simulink model "TestingFile1"  (R2022b)
settings: Solver=VariableStepAuto  StartTime=0.0  StopTime=24  FixedStep=5e-9  MaxStep=0.01  RelTol=1e-3  AbsTol=1e-6
undefined symbols (not defined in the file): Acid, Lead
libraries: spsSeriesRLCBranchLib x24, spsCurrentMeasurementLib x19, spsIdealSwitchLib x10, spsMosfetLib x6, spsPWMGeneratorDCDCLib x5, spsDiodeLib x4, spsBatteryLib x2, slpidlib x2, spsIGBTLib x2, spsPVArrayLib x2, spsVoltageMeasurementLib x2, spspowerguiLib x1
(part 1 of 2)
settings Model: Creator=Haroon  LastModifiedBy=Haroon

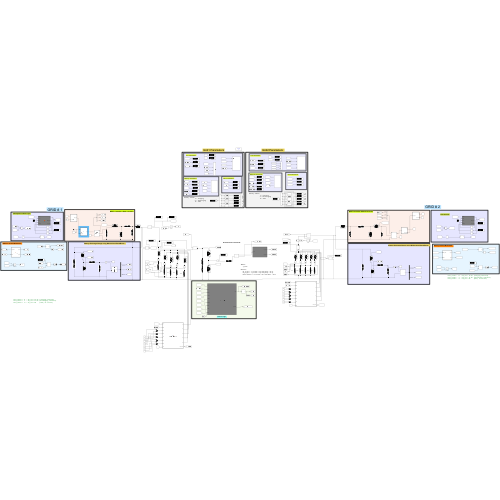
[thumbnail: Simulink's stored preview of the top-level diagram]
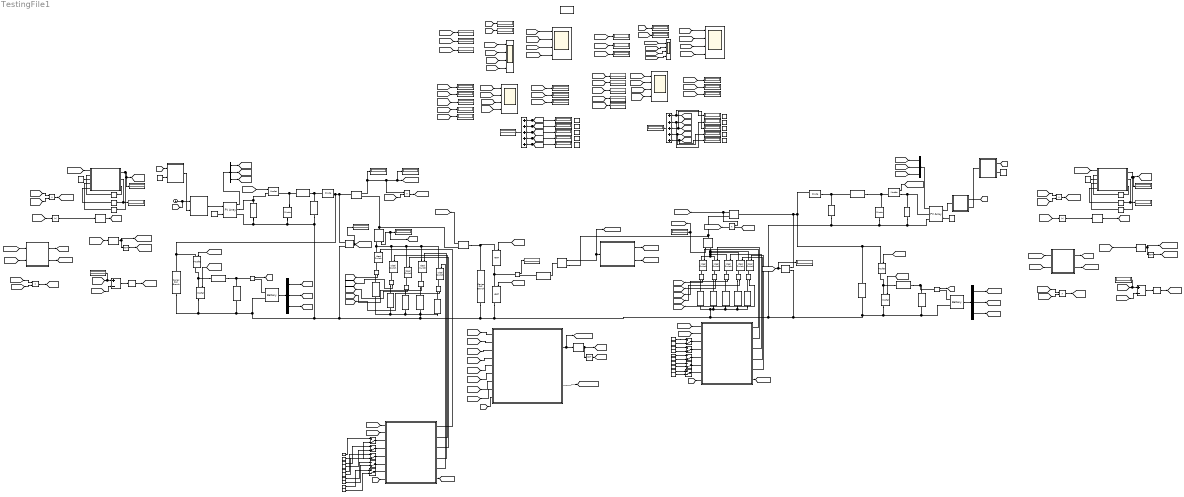
== system TestingFile1 ==
  note: Battery Status:
      | 1 = Charging
      | -1 = Discharging
      | 0 = Idle
  note: INPUTS:
      | I_flow
      |
      | OUTPUTS:
      | G1_to_G2 = 1 [I-flow > 0] and [Duty > 0.5]
      | G2_to_G1 = 1 [I-flow < 0] and [Duty < 0.5]
      | Both outputs = 0 [I-flow = 0] and [Duty = 0.5]
  note: batt_status = +1 → Vb_ref = 14.4V (charging reference)
      | batt_status = -1 → Vb_ref = 11.0V (discharging reference)
      | batt_status = 0 → Ib_ref = 0A (idle, no current)
  note: GRID # 1
  note: Control Logic
  note: Biredictional converter
  note: MPPT Controller - Buck converter
  note: Battery's Control Mechanism
  note: Battery Discharge/Charge using Bidirectional Buck/Boost Converter
  note: PV1 Parameters
  note: P&O Algorithm / MPPT Logic
  note: Battery1 Parameters
  note: Bus1 Parameters
  note: P&O Algorithm
  note: Battery2 Parameters
  note: PV2 Parameters
  note: Bus2 Parameters
  note: GRID # 2
  note: Grid1 Parameters
  note: Grid2 Parameters
  note: Battery's Control Mechanism
  note: batt_status = +1 → Vb_ref = 14.4V (charging reference)
      | batt_status = -1 → Vb_ref = 11.0V (discharging reference)
      | batt_status = 0 → Ib_ref = 0A (idle, no current)
  note: Battery Status:
      | 1 = Charging
      | -1 = Discharging
      | 0 = Idle
  note: Battery Discharge/Charge using Bidirectional Buck/Boost Converter
  note: MPPT Controller & Buck converter
  Abs : Abs  SaturateOnIntegerOverflow=off
  Abs2 : Abs  SaturateOnIntegerOverflow=off
  Add1 : Sum  Inputs=+-
  Add2 : Sum  Inputs=+++++
  Add3 : Sum  Inputs=+++++
  Add4 : Sum  Inputs=+-
  Battery : spsBatteryLib/Battery  BatType=Lead-Acid  ShowTempParam=off  ThermalPreset=no  ShowAgeParam=off  NomV=12  NomQ=0.01389  SOC=70  Batt_Tr=0.5  PresetModel=off  MaxQ=0.01389  MinV=10.5  FullV=14.4  Dis_rate=5  R=0.1  Normal_OP=0.01389  expZone="[12.2     0.001389]"  current=[6.5 13 32.5]  Units=Time  Tci=20  NomT=20  T2=-30  MaxQ2=4.8  FullV2=7.1  Normal_OP2=5.655  expZone2="[6.58           1]"  Rca=0.6  ti=2000  Dp=0  Neq0=0  Tsim=1e6  Ta1=25  Qeol=5.4*0.9  Reol=0.013333*1.2  Char_age=[2.3478, 3]  Dis_age=[2.3478, 10]  N1=1500  N2=10500  N3=1000  N4=1400  Ta2=45  N5=950
  Battery1 : spsBatteryLib/Battery  BatType=Lead-Acid  ShowTempParam=off  ThermalPreset=no  ShowAgeParam=off  NomV=12  NomQ=0.01389  SOC=70  Batt_Tr=0.5  PresetModel=off  MaxQ=0.01389  MinV=10.5  FullV=14.4  Dis_rate=5  R=0.1  Normal_OP=0.01389  expZone="[12.2     0.001389]"  current=[6.5 13 32.5]  Units=Time  Tci=20  NomT=20  T2=-30  MaxQ2=4.8  FullV2=7.1  Normal_OP2=5.655  expZone2="[6.58           1]"  Rca=0.6  ti=2000  Dp=0  Neq0=0  Tsim=1e6  Ta1=25  Qeol=5.4*0.9  Reol=0.013333*1.2  Char_age=[2.3478, 3]  Dis_age=[2.3478, 10]  N1=1500  N2=10500  N3=1000  N4=1400  Ta2=45  N5=950
  Bus Selector : BusSelector  OutputSignals=Current (A),Voltage (V),SOC (%)
  Bus Selector1 : BusSelector  OutputSignals=V_PV,I_PV,Irradiance (W/m2)
  Bus Selector2 : BusSelector  OutputSignals=V_PV,I_PV,Irradiance (W/m2)
  Bus Selector3 : BusSelector  OutputSignals=Current (A),Voltage (V),SOC (%)
  Clock : Clock
  Constant{1,5,10,12,14,16..17,19,21,24} (10 alike) : Constant  Value=0
  Constant{4,6,11,13,15,18,20,22..23,25} (10 alike) : Constant
  Constant2 : Constant  Value=25
  Constant7 : Constant  Value=25
  Constant8 : Constant  Value=1000
  Constant9 : Constant  Value=1000
  Current Measurement{,1..18} (19 alike) : spsCurrentMeasurementLib/Current Measurement  PhasorSimulation=off  OutputType=Complex  PSBequivalent=0
  Diode{,1..3} (4 alike) : spsDiodeLib/Diode  Ron=0.001  Lon=0  Vf=0.8  IC=0  UseSnubber=0  Rs=500  Cs=250e-9  Measurements=on
  Discrete PID Controller1 : slpidlib/PID Controller  Controller=PI  Form=Parallel  TimeDomain=Discrete-time  UseExternalTs=off  SampleTime=50e-6  IntegratorMethod=Forward Euler  FilterMethod=Forward Euler  ControllerParametersSource=internal  P=0.3  I=0.03  UseKiTs=off  D=0  N=100  UseFilter=on  TunerSelectOption=Transfer Function Based (PID Tuner App)  InitialConditionSource=internal  InitialConditionForIntegrator=0.5  InitialConditionForFilter=0  DifferentiatorICPrevScaledInput=0  ExternalReset=none  TrackingMode=off  Kt=1  LimitOutput=on  SatLimitsSource=internal  UpperSaturationLimit=0.95  LowerSaturationLimit=0.05  LinearizeAsGain=on  AntiWindupMode=back-calculation  Kb=1  LimitIntegrator=off  UpperIntegratorSaturationLimit=inf  LowerIntegratorSaturationLimit=-inf  POutMin=[]  POutMax=[]  IOutMin=[]  IOutMax=[]  DOutMin=[]  DOutMax=[]  NOutMin=[]  NOutMax=[]  SumOutMin=[]  SumOutMax=[]  SaturationOutMin=[]  SaturationOutMax=[]  PParamMin=[]  PParamMax=[]  IParamMin=[]  IParamMax=[]  DParamMin=[]  DParamMax=[]  NParamMin=[]  NParamMax=[]  KbParamMin=[]  KbParamMax=[]  KtParamMin=[]  KtParamMax=[]  KbOutMin=[]  KbOutMax=[]  KtOutMin=[]  KtOutMax=[]  IntegratorOutMin=[]  IntegratorOutMax=[]  FilterOutMin=[]  FilterOutMax=[]  SumI1OutMin=[]  SumI1OutMax=[]  SumI2OutMin=[]  SumI2OutMax=[]  SumI3OutMin=[]  SumI3OutMax=[]  SumI4OutMin=[]  SumI4OutMax=[]  SumDOutMin=[]  SumDOutMax=[]  DifferentiatorOutMin=[]  DifferentiatorOutMax=[]  FilterDiffOutCoefMin=[]  FilterDiffOutCoefMax=[]  ReciprocalOutMin=[]  ReciprocalOutMax=[]  SumDenOutMin=[]  SumDenOutMax=[]  SumNumOutMin=[]  SumNumOutMax=[]  DivideOutMin=[]  DivideOutMax=[]  UdiffTsProdOutMin=[]  UdiffTsProdOutMax=[]  NTsProdOutMin=[]  NTsProdOutMax=[]  UintegralTsProdOutMin=[]  UintegralTsProdOutMax=[]  UngainTsProdOutMin=[]  UngainTsProdOutMax=[]  ClampingZeroOutDataTypeStr=Inherit: Inherit via back propagation  ClampingZeroOutMin=[]  ClampingZeroOutMax=[]  FilterDenConstantOutDataTypeStr=Inherit: Inherit via back propagation  FilterDenConstantOutMin=[]  FilterDenConstantOutMax=[]  PCopyOutDataTypeStr=Inherit: Inherit via back propagation  PCopyOutMin=[]  PCopyOutMax=[]  NCopyOutDataTypeStr=Inherit: Inherit via back propagation  NCopyOutMin=[]  NCopyOutMax=[]  IntegratorContinuousStateAttributes=''  IntegratorStateMustResolveToSignalObject=off  IntegratorRTWStateStorageClass=Auto  FilterContinuousStateAttributes=''  FilterStateMustResolveToSignalObject=off  FilterRTWStateStorageClass=Auto  ParallelPVariant=InternalParameters  IdealPVariant=Disabled  IVariant=InternalParameters  DVariant=Disabled  IntegratorVariant=Discrete  SatVariant=Enabled  AWVariant=BackCalculation  PCopyVariant=Disabled  TRVariant=Disabled  FdbkBlocksVariant=Forward  IdealPFdbkVariant=Disabled  SatFdbkVariant=Disabled  DerivativeFilterVariant=Disabled  NVariant=Disabled  NCopyVariant=Disabled_SignalSpec  FilterICVariant=Disabled  IntegratorICVariant=InternalICs  ExternalResetVariant=Disabled  TRSumVariant=Passthrough  SumFdbkVariant=Disabled  SumVariant=Sum_PI  TsampFilterVariant=InternalTs  TsampNgainVariant=Passthrough  TsampIntegralVariant=Passthrough  ExternalSaturationOutDataTypeStr=Inherit: Same as second input
      settings: LibrarySourceBlock=simulink/Discrete/Discrete PID Controller
  Discrete PID Controller4 : slpidlib/PID Controller  Controller=PI  Form=Parallel  TimeDomain=Discrete-time  UseExternalTs=off  SampleTime=50e-6  IntegratorMethod=Forward Euler  FilterMethod=Forward Euler  ControllerParametersSource=internal  P=0.3  I=0.03  UseKiTs=off  D=0  N=100  UseFilter=on  TunerSelectOption=Transfer Function Based (PID Tuner App)  InitialConditionSource=internal  InitialConditionForIntegrator=0.5  InitialConditionForFilter=0  DifferentiatorICPrevScaledInput=0  ExternalReset=none  TrackingMode=off  Kt=1  LimitOutput=on  SatLimitsSource=internal  UpperSaturationLimit=0.95  LowerSaturationLimit=0.05  LinearizeAsGain=off  AntiWindupMode=back-calculation  Kb=1  LimitIntegrator=on  UpperIntegratorSaturationLimit=Inf  LowerIntegratorSaturationLimit=-Inf  POutMin=[]  POutMax=[]  IOutMin=[]  IOutMax=[]  DOutMin=[]  DOutMax=[]  NOutMin=[]  NOutMax=[]  SumOutMin=[]  SumOutMax=[]  SaturationOutMin=[]  SaturationOutMax=[]  PParamMin=[]  PParamMax=[]  IParamMin=[]  IParamMax=[]  DParamMin=[]  DParamMax=[]  NParamMin=[]  NParamMax=[]  KbParamMin=[]  KbParamMax=[]  KtParamMin=[]  KtParamMax=[]  KbOutMin=[]  KbOutMax=[]  KtOutMin=[]  KtOutMax=[]  IntegratorOutMin=[]  IntegratorOutMax=[]  FilterOutMin=[]  FilterOutMax=[]  SumI1OutMin=[]  SumI1OutMax=[]  SumI2OutMin=[]  SumI2OutMax=[]  SumI3OutMin=[]  SumI3OutMax=[]  SumI4OutMin=[]  SumI4OutMax=[]  SumDOutMin=[]  SumDOutMax=[]  DifferentiatorOutMin=[]  DifferentiatorOutMax=[]  FilterDiffOutCoefMin=[]  FilterDiffOutCoefMax=[]  ReciprocalOutMin=[]  ReciprocalOutMax=[]  SumDenOutMin=[]  SumDenOutMax=[]  SumNumOutMin=[]  SumNumOutMax=[]  DivideOutMin=[]  DivideOutMax=[]  UdiffTsProdOutMin=[]  UdiffTsProdOutMax=[]  NTsProdOutMin=[]  NTsProdOutMax=[]  UintegralTsProdOutMin=[]  UintegralTsProdOutMax=[]  UngainTsProdOutMin=[]  UngainTsProdOutMax=[]  ClampingZeroOutDataTypeStr=Inherit: Inherit via back propagation  ClampingZeroOutMin=[]  ClampingZeroOutMax=[]  FilterDenConstantOutDataTypeStr=Inherit: Inherit via back propagation  FilterDenConstantOutMin=[]  FilterDenConstantOutMax=[]  PCopyOutDataTypeStr=Inherit: Inherit via back propagation  PCopyOutMin=[]  PCopyOutMax=[]  NCopyOutDataTypeStr=Inherit: Inherit via back propagation  NCopyOutMin=[]  NCopyOutMax=[]  IntegratorContinuousStateAttributes=''  IntegratorStateMustResolveToSignalObject=off  IntegratorRTWStateStorageClass=Auto  FilterContinuousStateAttributes=''  FilterStateMustResolveToSignalObject=off  FilterRTWStateStorageClass=Auto  ParallelPVariant=InternalParameters  IdealPVariant=Disabled  IVariant=InternalParameters  DVariant=Disabled  IntegratorVariant=Discrete  SatVariant=Enabled  AWVariant=BackCalculation  PCopyVariant=Disabled  TRVariant=Disabled  FdbkBlocksVariant=Forward  IdealPFdbkVariant=Disabled  SatFdbkVariant=Disabled  DerivativeFilterVariant=Disabled  NVariant=Disabled  NCopyVariant=Disabled_SignalSpec  FilterICVariant=Disabled  IntegratorICVariant=InternalICs  ExternalResetVariant=Disabled  TRSumVariant=Passthrough  SumFdbkVariant=Disabled  SumVariant=Sum_PI  TsampFilterVariant=InternalTs  TsampNgainVariant=Passthrough  TsampIntegralVariant=Passthrough  ExternalSaturationOutDataTypeStr=Inherit: Same as second input
      settings: LibrarySourceBlock=simulink/Discrete/Discrete PID Controller
  Display{,1..5,8..16,18..19,21..31,36..48} (41 alike) : Display
  Goto29 : Goto
  IGBT2 : spsIGBTLib/IGBT  Ron=0.001  Lon=0  Vf=1  Tf=1e-6  Tt=2e-6  IC=0  Rs=1e5  Cs=inf  Measurements=on
  IGBT3 : spsIGBTLib/IGBT  Ron=0.001  Lon=0  Vf=1  Tf=1e-6  Tt=2e-6  IC=0  Rs=1e5  Cs=inf  Measurements=on
  I_PV : Display
  I_PV1 : Display
  Ideal Switch{,1..9} (10 alike) : spsIdealSwitchLib/Ideal Switch  Ron=0.001  Lon=0  IC=0  Rs=1e5  Cs=inf  Measurements=on
  Irradiance : Display
  Irradiance1 : Display
  Lamp{1..10} (10 alike) : LampBlock  LabelPosition=Hide
  Logical Operator : Logic  Operator=NOT  AllPortsSameDT=off  OutDataTypeStr=boolean
  Logical Operator2 : Logic  Operator=NOT  AllPortsSameDT=off  OutDataTypeStr=boolean
  Logical Operator3 : Logic  Operator=NOT  AllPortsSameDT=off  OutDataTypeStr=boolean
  MATLAB Function : MATLAB Function  TreatAsAtomicUnit=on
  MATLAB Function1 : MATLAB Function  TreatAsAtomicUnit=on
  MATLAB Function10 : MATLAB Function  TreatAsAtomicUnit=on
  MATLAB Function11 : MATLAB Function  TreatAsAtomicUnit=on
  MATLAB Function2 : MATLAB Function  TreatAsAtomicUnit=on
  MATLAB Function3 : MATLAB Function  TreatAsAtomicUnit=on
  MATLAB Function4 : MATLAB Function  TreatAsAtomicUnit=on
  MATLAB Function5 : MATLAB Function  TreatAsAtomicUnit=on
  MATLAB Function6 : MATLAB Function  TreatAsAtomicUnit=on
  MATLAB Function7 : MATLAB Function  TreatAsAtomicUnit=on
  MATLAB Function8 : MATLAB Function  TreatAsAtomicUnit=on
  MATLAB Function9 : MATLAB Function  TreatAsAtomicUnit=on
  Manual Switch{,1..9} (10 alike) : ManualSwitch  CurrentSetting=0
  Memory{,1,3..4} (4 alike) : Memory
  Memory2 : Memory  InitialCondition=0.5
  Memory5 : Memory  InitialCondition=0.5
  Mosfet{,1..5} (6 alike) : spsMosfetLib/Mosfet  Ron=0.1  Lon=0  Rd=0.01  Vfd=0  IC=0  Rs=1e5  Cs=inf  Measurements=on
  PV Array : spsPVArrayLib/PV Array  Npar=1  Nser=1  PlotType=array @ 25 deg.C & specified irradiances  S_vec="[ 1000  500  100 0 ]"  Temp_C_vec="[ 45 25  ]"  ModuleName=User-defined  PlotWhenSelected=off  Pm=262.6404  Ncell=72  Voc=26.7  Isc=13.97  Vm=22.22  Im=11.82  beta_Voc_pc=-0.37  alpha_Isc_pc=0.06  beta_Voc=-0.09879  alpha_Isc=0.008382  IL=14.0891  I0=6.4727e-10  nI=0.61024  Rsh=13.454  Rs=0.082721  RobustModel=off  RobustCellTemperature=313.3991  BAL=on  Tc=1e-6  Tfilter=5e-5
  PV Array1 : spsPVArrayLib/PV Array  Npar=1  Nser=1  PlotType=array @ 1000 W/m2 & specified temperatures  S_vec="[ 1000  500  100 ]"  Temp_C_vec="[ 45 25  ]"  ModuleName=User-defined  PlotWhenSelected=off  Pm=262.6404  Ncell=72  Voc=26.7  Isc=13.97  Vm=22.22  Im=11.82  beta_Voc_pc=-0.355  alpha_Isc_pc=0.06  beta_Voc=-0.094785  alpha_Isc=0.008382  IL=14.0358  I0=3.7786e-10  nI=0.59666  Rsh=13.8554  Rs=0.087929  RobustModel=off  RobustCellTemperature=313.3991  BAL=on  Tc=1e-6  Tfilter=5e-5
  PWM Generator (DC-DC) : spsPWMGeneratorDCDCLib/PWM Generator (DC-DC)  Fsw=5000  Ts=0
  PWM Generator (DC-DC)1 : spsPWMGeneratorDCDCLib/PWM Generator (DC-DC)  Fsw=20000  Ts=0
  PWM Generator (DC-DC)2 : spsPWMGeneratorDCDCLib/PWM Generator (DC-DC)  Fsw=5000  Ts=0
  PWM Generator (DC-DC)3 : spsPWMGeneratorDCDCLib/PWM Generator (DC-DC)  Fsw=20000  Ts=0
  PWM Generator (DC-DC)5 : spsPWMGeneratorDCDCLib/PWM Generator (DC-DC)  Fsw=5000  Ts=0
  P_Bus2 : Product
  P_PV : Display
  P_PV1 : Display
  P_battery1 : Product
  P_battery2 : Product
  P_bus1 : Product
  Ppv1 : Product
  Ppv2 : Product
  Pulse Generator : DiscretePulseGenerator  PulseType=Time based  Period=0.005  PulseWidth=99.9999
  Pulse Generator1 : DiscretePulseGenerator  PulseType=Time based  Period=0.005  PulseWidth=99.9999
  Scope{,1..5} (6 alike) : Scope  NumInputPorts=4
  Series RLC Branch : spsSeriesRLCBranchLib/Series RLC Branch  LConnTagsString=__new0  RConnTagsString=__new0  BranchType=RC  Resistance=1e-4  Inductance=1e-3  SetiL0=off  InitialCurrent=0  Capacitance=680e-6  Setx0=off  InitialVoltage=0  Measurements=None
  Series RLC Branch1 : spsSeriesRLCBranchLib/Series RLC Branch  LConnTagsString=__new0  RConnTagsString=__new0  BranchType=RL  Resistance=1e-4  Inductance=13e-3  SetiL0=off  InitialCurrent=0  Capacitance=1e-6  Setx0=off  InitialVoltage=0  Measurements=None
  Series RLC Branch11 : spsSeriesRLCBranchLib/Series RLC Branch  LConnTagsString=__new0  RConnTagsString=__new0  BranchType=RC  Resistance=1e-4  Inductance=1e-3  SetiL0=off  InitialCurrent=0  Capacitance=1000e-6  Setx0=off  InitialVoltage=0  Measurements=None
  Series RLC Branch12 : spsSeriesRLCBranchLib/Series RLC Branch  LConnTagsString=__new0  RConnTagsString=__new0  BranchType=RL  Resistance=1e-4  Inductance=13e-3  SetiL0=off  InitialCurrent=0  Capacitance=1e-6  Setx0=off  InitialVoltage=0  Measurements=None
  Series RLC Branch13 : spsSeriesRLCBranchLib/Series RLC Branch  LConnTagsString=__new0  RConnTagsString=__new0  BranchType=RC  Resistance=1e-4  Inductance=1e-3  SetiL0=off  InitialCurrent=0  Capacitance=20e-6  Setx0=off  InitialVoltage=0  Measurements=None
  Series RLC Branch14 : spsSeriesRLCBranchLib/Series RLC Branch  LConnTagsString=__new0  RConnTagsString=__new0  BranchType=RL  Resistance=1  Inductance=1e-3  SetiL0=off  InitialCurrent=0  Capacitance=1e-6  Setx0=off  InitialVoltage=0  Measurements=None
  Series RLC Branch2 : spsSeriesRLCBranchLib/Series RLC Branch  LConnTagsString=__new0  RConnTagsString=__new0  BranchType=RC  Resistance=1e-4  Inductance=1e-3  SetiL0=off  InitialCurrent=0  Capacitance=100e-6  Setx0=off  InitialVoltage=0  Measurements=None
  Series RLC Branch24 : spsSeriesRLCBranchLib/Series RLC Branch  LConnTagsString=__new0  RConnTagsString=__new0  BranchType=RL  Resistance=0.01  Inductance=24e-6  SetiL0=off  InitialCurrent=0  Capacitance=1e-6  Setx0=off  InitialVoltage=0  Measurements=None
  Series RLC Branch3 : spsSeriesRLCBranchLib/Series RLC Branch  LConnTagsString=__new0  RConnTagsString=__new0  BranchType=RC  Resistance=0.001  Inductance=1e-3  SetiL0=off  InitialCurrent=0  Capacitance=400e-6  Setx0=off  InitialVoltage=0  Measurements=None
  Series RLC Branch4 : spsSeriesRLCBranchLib/Series RLC Branch  LConnTagsString=__new0  RConnTagsString=__new0  BranchType=RL  Resistance=0.01  Inductance=24e-6  SetiL0=off  InitialCurrent=0  Capacitance=1e-6  Setx0=off  InitialVoltage=0  Measurements=None
  Series RLC Branch5 : spsSeriesRLCBranchLib/Series RLC Branch  LConnTagsString=__new0  RConnTagsString=__new0  BranchType=RC  Resistance=0.01  Inductance=1e-3  SetiL0=off  InitialCurrent=0  Capacitance=97e-6  Setx0=off  InitialVoltage=0  Measurements=None
  Series RLC Branch6 : spsSeriesRLCBranchLib/Series RLC Branch  LConnTagsString=__new0  RConnTagsString=__new0  BranchType=RC  Resistance=1  Inductance=1e-3  SetiL0=off  InitialCurrent=0  Capacitance=1e-6  Setx0=off  InitialVoltage=0  Measurements=None
  Series RLC Branch7 : spsSeriesRLCBranchLib/Series RLC Branch  LConnTagsString=__new0  RConnTagsString=__new0  BranchType=RC  Resistance=0.001  Inductance=1e-3  SetiL0=off  InitialCurrent=0  Capacitance=400e-6  Setx0=off  InitialVoltage=0  Measurements=None
  Series RLC Branch9 : spsSeriesRLCBranchLib/Series RLC Branch  LConnTagsString=__new0  RConnTagsString=__new0  BranchType=RC  Resistance=0.01  Inductance=1e-3  SetiL0=off  InitialCurrent=0  Capacitance=97e-6  Setx0=off  InitialVoltage=0  Measurements=None
  Stage : Display
  Stage1 : Display
  V_PV : Display
  V_PV1 : Display
  Voltage Measurement : spsVoltageMeasurementLib/Voltage Measurement  PhasorSimulation=off  OutputType=Complex  PSBequivalent=0
  Voltage Measurement1 : spsVoltageMeasurementLib/Voltage Measurement  PhasorSimulation=off  OutputType=Complex  PSBequivalent=0
  bulb{11..12,21..22} (4 alike) : spsSeriesRLCBranchLib/Series RLC Branch  LConnTagsString=__new0  RConnTagsString=__new0  BranchType=R  Resistance=7.2  Inductance=1e-3  SetiL0=off  InitialCurrent=0  Capacitance=1e-6  Setx0=off  InitialVoltage=0  Measurements=None
  fan{11..12,21..22} (4 alike) : spsSeriesRLCBranchLib/Series RLC Branch  LConnTagsString=__new0  RConnTagsString=__new0  BranchType=R  Resistance=2.4  Inductance=1e-3  SetiL0=off  InitialCurrent=0  Capacitance=1e-6  Setx0=off  InitialVoltage=0  Measurements=None
  powergui : spspowerguiLib/powergui  Priority=1  SimulationMode=Discrete  SampleTime=1  frequency=60  Iterations=50  frequencyindice=0  Pbase=100e6  ErrMax=1e-4  UnitsV=kV  UnitsW=MW  buscounter=0  FunctionMessages=off  echomessages=off  EnableUseOfTLC=off  CurrentSourceSwitches=off  DisableSnubberDevices=off  DisableRonSwitches=off  DisableVfSwitches=off  DisplayEquations=off  AutomaticDiscreteSolvers=off  SolverType=Tustin/Backward Euler (TBE)  Interpol=off  ExternalGateDelay=off  methode=off  Ts=100  x0status=blocks  SPID=on  SwTol=0  HookPort=off  NonlinearTolerance=1e-4  nMaxIteration=100  ContinueOnMaxIteration=off  RestoreLinks=warning  ResistiveCurrentMeasurement=off  Frange=[0:2:500]  Ylog=off  Xlog=on  ShowGrid=off  save=off  variable=ZData  structure=0  ZoomFFT=off  StartTime=0.0  cycles=1  DisplayStyle=1  fundamental=60  FreqAxis=off  MaxFrequency=1000  frequencyindicesteady=1  RmsSteady=1  display=off
  pump : spsSeriesRLCBranchLib/Series RLC Branch  LConnTagsString=__new0  RConnTagsString=__new0  BranchType=R  Resistance=1.44  Inductance=1e-3  SetiL0=off  InitialCurrent=0  Capacitance=1e-6  Setx0=off  InitialVoltage=0  Measurements=None
  pump1 : spsSeriesRLCBranchLib/Series RLC Branch  LConnTagsString=__new0  RConnTagsString=__new0  BranchType=R  Resistance=1.44  Inductance=1e-3  SetiL0=off  InitialCurrent=0  Capacitance=1e-6  Setx0=off  InitialVoltage=0  Measurements=None
  wires:
  [Vpv_Grid1] -> Ppv1/1
  MATLAB Function/3(Pold_out) -> Memory/1
  MATLAB Function/2(Stage_out) -> Stage/1, Memory1/1
  Memory/1 -> MATLAB Function/2(P_old)
  [Ipv_Grid1] -> Ppv1/2
  Current Measurement/1 -> [I_bat1]
  PV Array/1 -> Bus Selector1/1
  MATLAB Function/1(Y) -> Memory2/1, [d_Grid1], Display4/1
  Ppv1/1 -> [P_new_Grid1]
  Pulse Generator/1 -> MATLAB Function/3(Delay)
  [SOC_Grid1] -> Display2/1
  [Vpv_Grid1] -> V_PV/1
  Memory2/1 -> MATLAB Function/4(Yin)
  [P_new_Grid1] -> P_PV/1
  [Ipv_Grid1] -> I_PV/1
  Battery/1 -> Bus Selector/1
  Constant2/1 -> PV Array/2
  Bus Selector1/1 -> [Vpv_Grid1]  "<V_PV>"
  [vb_Grid1] -> Display/1
  Bus Selector1/2 -> [Ipv_Grid1]  "<I_PV>"
  Bus Selector/3 -> [SOC_Grid1]  "<SOC (%)>"
  Bus Selector/2 -> [vb_Grid1]  "<Voltage (V)>"
  Bus Selector/1 -> [ib_Grid1]  "<Current (A)>"
  Memory1/1 -> MATLAB Function/5(Stage_in)
  [ib_Grid1] -> Display1/1
  Bus Selector2/1 -> [Vpv_Grid2]  "<V_PV>"
  Constant7/1 -> PV Array1/2
  PV Array1/1 -> Bus Selector2/1
  Bus Selector2/2 -> [Ipv_Grid2]  "<I_PV>"
  Bus Selector3/1 -> [ib_Grid2]  "<Current (A)>"
  Bus Selector3/3 -> [SOC_Grid2]  "<SOC (%)>"
  Current Measurement1/1 -> [I_bat2]
  Bus Selector3/2 -> [vb_Grid2]  "<Voltage (V)>"
  Battery1/1 -> Bus Selector3/1
  Current Measurement2/1 -> Display10/1, [I_boost_Grid1], P_bus1/1, Display11/1
  P_bus1/1 -> [PLoad_Grid1]
  Current Measurement3/1 -> [I1_total], Display3/1
  Current Measurement4/1 -> Goto29/1
  Current Measurement5/1 -> Display5/1
  [s_p_Grid_X] -> IGBT2/1
  [s_n_Grid_X] -> IGBT3/1
  Current Measurement6/1 -> [I_Grid1_to_Grid2], MATLAB Function1/1(I_flow)
  MATLAB Function1/2(G2_to_G1) -> [Grid2to1]
  MATLAB Function1/1(G1_to_G2) -> [Grid1to2]
  Current Measurement7/1 -> [I2_total], Display8/1
  Current Measurement8/1 -> [I_boost_Grid2], P_Bus2/1
  P_Bus2/1 -> [PLoad_Grid2]
  [P_new_Grid1] -> MATLAB Function/1(P_new)
  [I_boost_Grid1] -> Display14/1
  [V_bus_Grid1] -> Display13/1
  [PLoad_Grid1] -> Display15/1
  Memory4/1 -> MATLAB Function3/5(Stage_in)
  Memory5/1 -> MATLAB Function3/4(Yin)
  [d_Grid2] -> Abs2/1
  Ppv2/1 -> [P_new_Grid2]
  MATLAB Function3/1(Y) -> Memory5/1, [d_Grid2], Display16/1
  Memory3/1 -> MATLAB Function3/2(P_old)
  Pulse Generator1/1 -> MATLAB Function3/3(Delay)
  [Ipv_Grid2] -> Ppv2/2
  [Vpv_Grid2] -> Ppv2/1
  MATLAB Function3/3(Pold_out) -> Memory3/1
  MATLAB Function3/2(Stage_out) -> Stage1/1, Memory4/1
  [P_new_Grid2] -> MATLAB Function3/1(P_new)
  [ib_Grid1] -> Display19/1, Add1/1
  [ib_ref_Grid1] -> Add1/2
  Add1/1 -> Discrete PID Controller1/1
  Discrete PID Controller1/1 -> [duty_B_Grid1]
  PWM Generator (DC-DC)3/1 -> Logical Operator/1, [s_p_Grid1]
  Logical Operator/1 -> [s_n_Grid1]
  [Vpv_Grid2] -> V_PV1/1
  [Ipv_Grid2] -> I_PV1/1
  [V_bus_Grid2] -> Display25/1
  [I_boost_Grid2] -> Display26/1
  [PLoad_Grid2] -> Display27/1
  [P_new_Grid2] -> P_PV1/1
  PWM Generator (DC-DC)5/1 -> Logical Operator3/1, [s_p_Grid_X]
  Logical Operator3/1 -> [s_n_Grid_X]
  [vb_Grid2] -> Display23/1
  [ib_Grid2] -> Display24/1
  [SOC_Grid2] -> Display28/1
  [Duty_Grid1] -> Mosfet4/1
  [Duty_Grid2] -> Mosfet5/1
  [d_Grid1] -> Abs/1
  Constant8/1 -> MATLAB Function4/2(G_meas)
  MATLAB Function4/1(day_type) -> MATLAB Function5/2(day_type)
  MATLAB Function5/1(G) -> PV Array/1
  Clock/1 -> [Clock], MATLAB Function5/1(t)
  [Clock] -> MATLAB Function6/1(t)
  Constant9/1 -> MATLAB Function6/2(G_meas)
  MATLAB Function7/1(G) -> PV Array1/1
  [Clock] -> MATLAB Function7/1(t)
  MATLAB Function6/1(day_type) -> MATLAB Function7/2(day_type)
  Bus Selector2/3 -> [Irr_Grid2]  "<Irradiance (W/m2)>"
  Bus Selector1/3 -> [Irr_Grid1]  "<Irradiance (W/m2)>"
  [Clock] -> MATLAB Function4/1(t)
  [V_bus_Grid1] -> MATLAB Function2/1(V1)
  [V_bus_Grid2] -> MATLAB Function2/2(V2)
  [SOC_Grid1] -> MATLAB Function2/3(SOC1)
  [SOC_Grid2] -> MATLAB Function2/4(SOC2)
  [PLoad_Grid1] -> MATLAB Function2/5(Pload1)
  [PLoad_Grid2] -> MATLAB Function2/6(Pload2)
  [P_new_Grid1] -> MATLAB Function2/7(PPV1)
  [P_new_Grid2] -> MATLAB Function2/8(PPV2)
  Manual Switch/1 -> MATLAB Function8/3(sw1)
  Manual Switch1/1 -> MATLAB Function8/4(sw2)
  Manual Switch2/1 -> MATLAB Function8/5(sw3)
  Manual Switch3/1 -> MATLAB Function8/6(sw4)
  Manual Switch4/1 -> MATLAB Function8/7(sw5)
  [P_new_Grid1] -> MATLAB Function8/1(P_pv)
  Constant14/1 -> Manual Switch4/1
  Constant15/1 -> Manual Switch4/2
  Constant12/1 -> Manual Switch3/1
  Constant13/1 -> Manual Switch3/2
  Constant10/1 -> Manual Switch2/1
  Constant11/1 -> Manual Switch2/2
  Constant5/1 -> Manual Switch1/1
  Constant6/1 -> Manual Switch1/2
  Constant1/1 -> Manual Switch/1
  Constant4/1 -> Manual Switch/2
  [Clock] -> MATLAB Function8/8(Hour)
  [SOC_Grid1] -> MATLAB Function8/2(SOC)
  MATLAB Function8/1(r1) -> Ideal Switch/1
  MATLAB Function8/2(r2) -> Ideal Switch1/1
  MATLAB Function8/3(r3) -> Ideal Switch2/1
  MATLAB Function8/4(r4) -> Ideal Switch3/1
  MATLAB Function8/5(r5) -> Ideal Switch4/1
  MATLAB Function8/6(batt_status) -> [Battery1_state]
  [Battery1_state] -> MATLAB Function9/1(batt_status)
  [SOC_Grid1] -> MATLAB Function9/2(SOC)
  MATLAB Function9/2(Ib_ref) -> [ib_ref_Grid1]
  MATLAB Function9/1(Vb_ref) -> [vb_ref_Grid1]
  MATLAB Function2/2(P_transfer) -> [P_trans]
  [Battery2_state] -> MATLAB Function10/1(batt_status)
  MATLAB Function10/1(Vb_ref) -> [vb_ref_Grid2]
  MATLAB Function10/2(Ib_ref) -> [ib_ref_Grid2]
  [SOC_Grid2] -> MATLAB Function10/2(SOC)
  PWM Generator (DC-DC)1/1 -> Logical Operator2/1, [s_p_Grid2]
  Add4/1 -> Discrete PID Controller4/1
  Discrete PID Controller4/1 -> [duty_B_Grid2]
  [ib_Grid2] -> Display18/1, Add4/1
  Logical Operator2/1 -> [s_n_Grid2]
  [ib_ref_Grid2] -> Add4/2
  [P_new_Grid2] -> MATLAB Function11/1(P_pv)
  [SOC_Grid2] -> MATLAB Function11/2(SOC)
  Constant22/1 -> Manual Switch9/2
  Constant19/1 -> Manual Switch8/1
  Constant17/1 -> Manual Switch7/1
  Manual Switch9/1 -> MATLAB Function11/7(sw5)
  Constant20/1 -> Manual Switch8/2
  Manual Switch8/1 -> MATLAB Function11/6(sw4)
  Constant18/1 -> Manual Switch7/2
  Manual Switch7/1 -> MATLAB Function11/5(sw3)
  Constant21/1 -> Manual Switch9/1
  Manual Switch6/1 -> MATLAB Function11/4(sw2)
  [Clock] -> MATLAB Function11/8(Hour)
  Constant23/1 -> Manual Switch5/2
  Constant25/1 -> Manual Switch6/2
  Constant16/1 -> Manual Switch5/1
  Constant24/1 -> Manual Switch6/1
  Manual Switch5/1 -> MATLAB Function11/3(sw1)
  MATLAB Function11/6(batt_status) -> [Battery2_state]
  Current Measurement9/1 -> [fan11]
  Current Measurement10/1 -> [bulb11]
  Current Measurement11/1 -> [pump]
  Current Measurement12/1 -> [fan12]
  Current Measurement13/1 -> [bulb12]
  Voltage Measurement/1 -> Display12/1, [V_bus_Grid1]
  [V_bus_Grid1] -> P_bus1/2
  MATLAB Function11/1(r1) -> Ideal Switch5/1
  MATLAB Function11/2(r2) -> Ideal Switch6/1
  MATLAB Function11/3(r3) -> Ideal Switch7/1
  MATLAB Function11/4(r4) -> Ideal Switch8/1
  MATLAB Function11/5(r5) -> Ideal Switch9/1
  Voltage Measurement1/1 -> Display9/1, [V_bus_Grid2]
  [V_bus_Grid2] -> P_Bus2/2
  [Clock] -> Display21/1
  [Clock] -> Display22/1
  [Irr_Grid2] -> Irradiance1/1
  [Irr_Grid1] -> Irradiance/1
  Current Measurement14/1 -> [fan21]
  Current Measurement15/1 -> [bulb21]
  Current Measurement16/1 -> [pump1]
  Current Measurement17/1 -> [fan22]
  Current Measurement18/1 -> [bulb22]
  [Battery2_state] -> Display41/1
  [Battery1_state] -> Display42/1
  [bulb11] -> Display45/1, Add3/2
  [pump] -> Display46/1, Add3/3
  [bulb12] -> Display48/1, Add3/5
  [fan11] -> Display44/1, Add3/1
  [fan12] -> Display47/1, Add3/4
  Add3/1 -> Display43/1
  Add2/1 -> Display29/1
  [bulb21] -> Display37/1, Add2/2
  [bulb22] -> Display40/1, Add2/5
  [fan22] -> Display39/1, Add2/4
  [pump1] -> Add2/3, Display38/1
  [fan21] -> Display36/1, Add2/1
  [Irr_Grid2] -> Scope/1
  [P_new_Grid2] -> Scope/2
  [ib_Grid2] -> P_battery2/2
  [vb_Grid2] -> P_battery2/1
  P_battery2/1 -> [P_battery2]
  [ib_Grid1] -> P_battery1/2
  [vb_Grid1] -> P_battery1/1
  P_battery1/1 -> [P_battery1]
  [P_battery1] -> Display30/1
  [P_battery2] -> Display31/1
  [P_battery2] -> Scope4/4
  [ib_Grid2] -> Scope4/3
  [vb_Grid2] -> Scope4/2
  [Battery2_state] -> Scope4/1
  [vb_Grid1] -> Scope2/2
  [P_battery1] -> Scope2/4
  [ib_Grid1] -> Scope2/3
  [Battery1_state] -> Scope2/1
  [P_battery2] -> Scope/3
  [PLoad_Grid2] -> Scope/4
  [PLoad_Grid1] -> Scope3/4
  [P_new_Grid1] -> Scope3/2
  [Irr_Grid1] -> Scope3/1
  [P_battery1] -> Scope3/3
  [s_p_Grid1] -> Mosfet/1
  [s_n_Grid1] -> Mosfet1/1
  [s_p_Grid2] -> Mosfet2/1
  [s_n_Grid2] -> Mosfet3/1
  [duty_B_Grid1] -> PWM Generator (DC-DC)3/1
  [duty_B_Grid2] -> PWM Generator (DC-DC)1/1
  PWM Generator (DC-DC)2/1 -> [Duty_Grid2]
  PWM Generator (DC-DC)/1 -> [Duty_Grid1]
  Abs/1 -> PWM Generator (DC-DC)/1
  Abs2/1 -> PWM Generator (DC-DC)2/1
  MATLAB Function2/1(duty) -> PWM Generator (DC-DC)5/1, [sharing_duty]
  [P_new_Grid1] -> Scope1/4
  [Vpv_Grid1] -> Scope1/3
  [Irr_Grid1] -> Scope1/1
  [Ipv_Grid1] -> Scope1/2
  [Irr_Grid2] -> Scope5/1
  [Ipv_Grid2] -> Scope5/2
  [Vpv_Grid2] -> Scope5/3
  [P_new_Grid2] -> Scope5/4
  [Clock] -> MATLAB Function2/9(Hour)
  connections:
  Current Measurement/LConn1 -- Series RLC Branch1/RConn1 -- Series RLC Branch2/LConn1
  Series RLC Branch1/LConn1 -- Mosfet1/LConn1 -- Mosfet/RConn1
  Diode2/RConn1 -- Mosfet4/RConn1 -- Series RLC Branch4/LConn1
  PV Array/RConn1 -- Mosfet4/LConn1 -- Series RLC Branch3/LConn1
  Battery/LConn1 -- Current Measurement/RConn1
  Voltage Measurement/LConn1 -- Mosfet/LConn1 -- Series RLC Branch/LConn1 -- Diode/RConn1 -- Current Measurement2/LConn1
  PV Array1/RConn1 -- Mosfet5/LConn1 -- Series RLC Branch7/LConn1
  Series RLC Branch12/LConn1 -- Mosfet3/LConn1 -- Mosfet2/RConn1
  Series RLC Branch13/LConn1 -- Series RLC Branch12/RConn1 -- Current Measurement1/LConn1
  Battery1/LConn1 -- Current Measurement1/RConn1
  Current Measurement3/LConn1 -- Current Measurement2/RConn1 -- Current Measurement4/RConn1
  Current Measurement4/LConn1 -- IGBT2/LConn1 -- Series RLC Branch6/LConn1
  Current Measurement5/LConn1 -- IGBT3/LConn1 -- IGBT2/RConn1
  Series RLC Branch14/LConn1 -- Current Measurement5/RConn1
  Current Measurement6/LConn1 -- Series RLC Branch14/RConn1
  Current Measurement6/RConn1 -- Current Measurement8/RConn1 -- Current Measurement7/LConn1
  Series RLC Branch11/LConn1 -- Current Measurement8/LConn1 -- Voltage Measurement1/LConn1 -- Diode3/RConn1 -- Mosfet2/LConn1
  Diode1/RConn1 -- Series RLC Branch24/RConn1 -- Mosfet5/RConn1
  Diode2/LConn1 -- bulb22/RConn1 -- fan22/RConn1 -- pump1/RConn1 -- bulb21/RConn1 -- fan21/RConn1 -- Voltage Measurement1/LConn2 -- Mosfet3/RConn1 -- Battery1/LConn2 -- Series RLC Branch13/RConn1 -- Series RLC Branch11/RConn1 -- Series RLC Branch9/RConn1 -- Series RLC Branch7/RConn1 -- PV Array1/RConn2 -- Diode1/LConn1 -- IGBT3/RConn1 -- Series RLC Branch6/RConn1 -- bulb12/RConn1 -- fan11/RConn1 -- bulb11/RConn1 -- pump/RConn1 -- fan12/RConn1 -- Voltage Measurement/LConn2 -- Battery/LConn2 -- Series RLC Branch/RConn1 -- Mosfet1/RConn1 -- Series RLC Branch2/RConn1 -- Series RLC Branch5/RConn1 -- PV Array/RConn2 -- Series RLC Branch3/RConn1
  Series RLC Branch4/RConn1 -- Diode/LConn1 -- Series RLC Branch5/LConn1
  Series RLC Branch24/LConn1 -- Diode3/LConn1 -- Series RLC Branch9/LConn1
  Current Measurement3/RConn1 -- Ideal Switch4/LConn1 -- Ideal Switch3/LConn1 -- Ideal Switch2/LConn1 -- Ideal Switch1/LConn1 -- Ideal Switch/LConn1
  Current Measurement9/LConn1 -- Ideal Switch/RConn1
  fan11/LConn1 -- Current Measurement9/RConn1
  Current Measurement10/LConn1 -- Ideal Switch1/RConn1
  Current Measurement11/LConn1 -- Ideal Switch2/RConn1
  Current Measurement12/LConn1 -- Ideal Switch3/RConn1
  Current Measurement13/LConn1 -- Ideal Switch4/RConn1
  Current Measurement10/RConn1 -- bulb11/LConn1
  Current Measurement11/RConn1 -- pump/LConn1
  Current Measurement12/RConn1 -- fan12/LConn1
  Current Measurement13/RConn1 -- bulb12/LConn1
  Current Measurement14/LConn1 -- Ideal Switch5/RConn1
  Ideal Switch5/LConn1 -- Ideal Switch6/LConn1 -- Ideal Switch7/LConn1 -- Ideal Switch8/LConn1 -- Ideal Switch9/LConn1 -- Current Measurement7/RConn1
  fan21/LConn1 -- Current Measurement14/RConn1
  Current Measurement15/LConn1 -- Ideal Switch6/RConn1
  Current Measurement16/LConn1 -- Ideal Switch7/RConn1
  Current Measurement17/LConn1 -- Ideal Switch8/RConn1
  Current Measurement18/LConn1 -- Ideal Switch9/RConn1
  bulb22/LConn1 -- Current Measurement18/RConn1
  Current Measurement17/RConn1 -- fan22/LConn1
  pump1/LConn1 -- Current Measurement16/RConn1
  bulb21/LConn1 -- Current Measurement15/RConn1

== matlab function TestingFile1/MATLAB Function7 ==
  data: t input; G output; day_type input
function G = irradiance_generator(t, day_type)
% Generates irradiance based on selected day type

T = (0:23);

G_summer = [ ...
    0 0 0 0 0 50 150 300 500 700 850 950 ...
    1000 980 900 750 600 400 200 80 0 0 0 0 ];

G_winter = [ ...
    0 0 0 0 0 0 0 50 150 300 450 600 ...
    700 650 500 350 200 80 0 0 0 0 0 0 ];

G_cloudy = [ ...
    0 0 0 0 0 0 60 120 250 400 300 450 ...
    500 350 420 280 180 90 30 0 0 0 0 0 ];

% Select profile
if day_type == 1
    G_table = G_summer;
elseif day_type == 2
    G_table = G_winter;
else
    G_table = G_cloudy;
end

% Time saturation
t = min(max(t,0), T(end));

% Interpolated irradiance
G = interp1(T, G_table, t);

== matlab function TestingFile1/MATLAB Function8 ==
  settings: updateMethod=DISCRETE  sampleTime=1
  data: P_pv input; SOC input; r1 output; r2 output; r3 output; r4 output; r5 output; batt_status output; sw1 input; sw2 input; sw3 input; sw4 input; sw5 input; Hour input
function [r1, r2, r3, r4, r5, batt_status] = nanogrid_optimization(P_pv, SOC, sw1, sw2, sw3, sw4, sw5, Hour)
% =========================================================================
%   MICROGRID OPTIMIZATION CONTROLLER  v5.0  — Simplified & Corrected
% =========================================================================
%
% SYSTEM:
%   PV      : 260W
%   Battery : 12V, 50Ah  |  Max I = 5A  |  Max P = 60W  |  Backup = 10hrs
%   Bus     : 12V DC
%
% LOADS:
%   r1 = Fan1   60W   CRITICAL
%   r2 = Bulb1  20W   CRITICAL
%   r3 = Pump  100W   Non-Critical  ← ALWAYS OFF during day
%   r4 = Fan2   60W   Non-Critical  ← ALWAYS OFF during day
%   r5 = Bulb2  20W   Non-Critical  ← ALWAYS OFF during day
%
% =========================================================================
%  SIMPLIFIED DAY RULES (your latest requirement)
% =========================================================================
%
%  During the day, there are only 3 things that matter — in this order:
%
%    PRIORITY 1 → Fan1  (critical, 60W)
%    PRIORITY 2 → Bulb1 (critical, 20W)
%    PRIORITY 3 → CHARGE BATTERY (60W = 5A)
%    NC LOADS   → ALWAYS SHED. No exceptions. They never run during day.
%
%  The battery SOC window is strictly maintained:
%    SOC must stay ABOVE 40%  (no deep discharge)
%    SOC must stay BELOW 90%  (no overcharge)
%
%  Battery charging happens whenever:
%    - SOC < 90%  AND  P_pv is available
%    - After Fan1 and Bulb1 are powered, remaining PV goes to battery
%
%  Battery discharging happens when:
%    - P_pv alone cannot power Fan1 and/or Bulb1
%    - SOC > 40% (safe to discharge)
%    - Battery fills ONLY the gap needed for critical loads
%    - NC loads are STILL not powered even during discharge
%
% =========================================================================
%  NIGHT RULES (unchanged)
% =========================================================================
%
%  PRIORITY 1 → Fan1 (if sw1=1)  → 60W = exactly 5A cap → alone, nothing else
%  PRIORITY 2 → If sw1=0: Bulb1 + Bulb2 only (40W = 3.33A, within cap)
%  Pump (r3) and Fan2 (r4) are NEVER allowed at night
%  SOC ≤ 40% at night → everything OFF (protect battery)
%
% =========================================================================
%  WHAT WAS WRONG IN v4.0 (explanation of bugs fixed here)
% =========================================================================
%
%  Bug 1 — Battery discharging in early simulation then going idle:
%    Root cause: Scenario D (discharge pass) was blocked by condition
%    (batt_status ~= 1). When SOC was between 40-90% and P_pv was low,
%    Scenario B set batt_status=1 (charging) even when P_pv couldn't
%    actually charge. This blocked the discharge path entirely, leaving
%    the battery idle instead of supporting critical loads.
%    Fix: Day logic is now a clean if-elseif chain. Discharge is handled
%    as its own first-class scenario, not a secondary pass.
%
%  Bug 2 — NC loads turning on during day:
%    Root cause: Step 4 in Scenario B allowed NC loads from "scraps"
%    after battery reservation. This violated the requirement.
%    Fix: NC loads (r3, r4, r5) are hardcoded to 0 in day mode.
%    They cannot turn on under any daytime condition.
%
%  Bug 3 — Battery staying idle when it should charge:
%    Root cause: After SOC rose above the old SOC_BATT_CRIT=70% threshold,
%    the code fell into Scenario C which kept battery idle even when SOC
%    was between 70-90% and PV had surplus.
%    Fix: Charging is attempted for ALL SOC values below SOC_HIGH=90%.
%    Any leftover PV after critical loads goes to battery, always.
%
% =========================================================================
% INPUTS:
%   P_pv    — Solar power (W)              Wiring: Vpv × Ipv
%   SOC     — Battery state of charge (%)  Wiring: Battery → BusSelector → SOC
%   sw1–sw5 — User switches (1=ON, 0=OFF)  Wiring: Constant blocks
%   Hour    — Hour of day 0–24             Wiring: Clock ÷ 3600
%
% OUTPUTS:
%   r1–r5       — Relay signals (1=ON, 0=OFF)
%   batt_status — +1=Charging | -1=Discharging | 0=Idle → feeds FUNC5
% =========================================================================

    %% ============================================================
    %  CONSTANTS
    % =============================================================

    % Load power [Fan1  Bulb1  Pump   Fan2   Bulb2]
    Load_W = [60,   20,    100,   60,    20  ];

    % SOC hard limits — the ONLY two SOC rules that matter now
    SOC_HIGH    = 90;   % Never charge above this  → stop charging at 90%
    SOC_LOW     = 40;   % Never discharge below this → stop discharging at 40%
    SOC_FLOOR   = 5;    % Absolute emergency cutoff (hardware protection)

    % Battery power — fixed at 5A × 12V = 60W in both directions
    BATT_W      = 60;   % Watts (= 5A × 12V)

    % Night window
    NIGHT_START = 20;   % 8 PM
    NIGHT_END   = 6;    % 6 AM

    %% ============================================================
    %  SETUP
    % =============================================================

    SW       = [sw1, sw2, sw3, sw4, sw5];
    is_Night = (Hour >= NIGHT_START) || (Hour < NIGHT_END);

    % Default outputs — safe starting state
    Relays      = [0, 0, 0, 0, 0];
    batt_status = 0;

    %% ============================================================
    %  NIGHT MODE
    % =============================================================

    if is_Night

        % ── Safety floor: SOC too low → protect battery ──────────
        if SOC <= SOC_LOW
            Relays      = [0, 0, 0, 0, 0];
            batt_status = 0;

        % ── Fan1 switch ON → Fan1 only (60W = entire 5A budget) ──
        elseif SW(1) == 1
            Relays(1)   = 1;    % Fan1 ON  — 60W
            % All others stay 0 — 5A cap is fully used by Fan1
            batt_status = -1;   % Discharging at 5A

        % ── Fan1 switch OFF → Bulb1 + Bulb2 only (max 40W) ──────
        else
            P_night = BATT_W;   % 60W budget available

            if SW(2) == 1 && P_night >= Load_W(2)   % Bulb1 = 20W
                Relays(2) = 1;
                P_night   = P_night - Load_W(2);
            end
            if SW(5) == 1 && P_night >= Load_W(5)   % Bulb2 = 20W
                Relays(5) = 1;
                P_night   = P_night - Load_W(5);
            end
            % Pump (r3) and Fan2 (r4) — forbidden at night, stay 0

            if any(Relays)
                batt_status = -1;   % Discharging
            else
                batt_status = 0;    % No loads on → idle
            end
        end

        % ── Twilight edge: PV trickling in → charge if possible ──
        if P_pv > 10 && SOC < SOC_HIGH
            Relays      = [0, 0, 0, 0, 0];  % Turn loads off, prioritize charging
            batt_status = 1;                  % Charging with twilight PV
        end

    end  % ── end night ──

    %% ============================================================
    %  DAY MODE
    %  NC loads (r3, r4, r5) are HARDCODED to 0 here.
    %  They cannot turn on under ANY daytime condition.
    %  Three scenarios only:
    %    DAY-1: Solar alone covers critical loads → charge with surplus
    %    DAY-2: Solar cannot cover critical loads → discharge fills gap
    %    DAY-3: SOC out of window → battery idle, solar only
    % =============================================================

    if ~is_Night

        % NC loads permanently OFF during day — no exceptions
        Relays(3) = 0;   % Pump  OFF
        Relays(4) = 0;   % Fan2  OFF
        Relays(5) = 0;   % Bulb2 OFF

        % Power needed for critical loads only
        P_crit_needed = (SW(1) * Load_W(1)) + (SW(2) * Load_W(2));
        % Max = 60+20 = 80W if both switched ON

        % ============================================================
        %  DAY SCENARIO 1: SOLAR ≥ CRITICAL LOADS
        %  P_pv can cover Fan1 + Bulb1 on its own.
        %  Any remaining PV after critical loads → battery charging.
        %  Charging happens for ALL SOC values between 40% and 90%.
        % ============================================================
        if P_pv >= P_crit_needed

            P_rem = P_pv;

            % Step 1: Fan1 from solar
            if SW(1) == 1
                Relays(1) = 1;
                P_rem     = P_rem - Load_W(1);
            end

            % Step 2: Bulb1 from solar
            if SW(2) == 1
                Relays(2) = 1;
                P_rem     = P_rem - Load_W(2);
            end

            % Step 3: Charge battery with ALL remaining solar
            %   - Only charge if SOC < 90%
            %   - Charge with whatever P_rem is available (up to 60W = 5A cap)
            %   - FUNC5 will handle the actual current limiting via PI controller
            if P_rem > 0 && SOC < SOC_HIGH
                batt_status = 1;    % CHARGING — any surplus goes to battery
            else
                batt_status = 0;    % SOC already full or no surplus
            end

        % ============================================================
        %  DAY SCENARIO 2: SOLAR < CRITICAL LOADS
        %  P_pv alone cannot power Fan1 + Bulb1.
        %  Battery discharges to fill the gap — max 60W (5A).
        %  Only fires if SOC > 40% (safe to discharge).
        %  NC loads are still OFF.
        % ============================================================
        elseif SOC > SOC_LOW

            % Combined power available = solar + battery discharge (max 60W)
            % Battery fills exactly the gap that solar cannot cover.
            % Total budget = P_pv + up to 60W from battery.
            % Example: P_pv=0W → 0+60=60W available → Fan1(60)=ON, Bulb1? 0W left → OFF
            % Example: P_pv=30W → 30+60=90W available → Fan1(60)=30W left → Bulb1(20)=ON
            P_available = P_pv + BATT_W;
            P_rem       = P_available;

            % Fan1 from combined source (solar + battery)
            if SW(1) == 1 && P_rem >= Load_W(1)
                Relays(1) = 1;
                P_rem     = P_rem - Load_W(1);
            end

            % Bulb1 from combined source
            if SW(2) == 1 && P_rem >= Load_W(2)
                Relays(2) = 1;
                P_rem     = P_rem - Load_W(2);
            end

            % Battery is discharging to support critical loads
            batt_status = -1;   % DISCHARGING

        % ============================================================
        %  DAY SCENARIO 3: SOC AT OR BELOW 40%
        %  Battery is empty — cannot discharge.
        %  Solar powers whatever critical loads it can alone.
        %  Battery stays idle to prevent deep discharge damage.
        % ============================================================
        else
            % SOC <= SOC_LOW (40%) — solar only, no battery

            P_rem = P_pv;

            if SW(1) == 1 && P_rem >= Load_W(1)
                Relays(1) = 1;
                P_rem     = P_rem - Load_W(1);
            end
            if SW(2) == 1 && P_rem >= Load_W(2)
                Relays(2) = 1;
                P_rem     = P_rem - Load_W(2);
            end

            batt_status = 0;    % IDLE — protecting battery from deep discharge
        end

    end  % ── end day ──

    %% ============================================================
    %  HARD SAFETY OVERRIDES
    %  Applied last, unconditionally, cannot be bypassed by any scenario.
    % =============================================================

    % OA: Absolute SOC floor — emergency stop
    if SOC <= SOC_FLOOR
        batt_status = 0;
    end

    % OB: Overcharge ceiling — never go above 100%
    if SOC >= 100
        batt_status = 0;
    end

    % OC: SOC hit 90% → stop charging immediately
    if SOC >= SOC_HIGH
        if batt_status == 1
            batt_status = 0;   % Charging was active — stop now
        end
    end

    % OD: SOC hit 40% → stop discharging immediately
    if SOC <= SOC_LOW
        if batt_status == -1
            batt_status = 0;   % Discharging was active — stop now
        end
    end

    % OE: No solar AND SOC at floor → cut everything
    if (P_pv < 5) && (SOC <= SOC_LOW)
        Relays      = [0, 0, 0, 0, 0];
        batt_status = 0;
    end

    % OF: Night + SOC at floor → cut everything
    if is_Night && (SOC <= SOC_LOW)
        Relays      = [0, 0, 0, 0, 0];
        batt_status = 0;
    end

    %% ============================================================
    %  ASSIGN OUTPUTS
    % =============================================================
    r1 = Relays(1);   % Fan1  — 60W  — CRITICAL
    r2 = Relays(2);   % Bulb1 — 20W  — CRITICAL
    r3 = Relays(3);   % Pump  — 100W — NC — always 0 during day
    r4 = Relays(4);   % Fan2  — 60W  — NC — always 0 during day
    r5 = Relays(5);   % Bulb2 — 20W  — NC — always 0 during day

end
